simulink library "Linkage_Uprights"  (R2025a)
settings: Solver=VariableStepAuto  StartTime=0.0  StopTime=10.0  RelTol=1e-3
undefined symbols (not defined in the file): acamber, atoe, axle_len, axle_mass, axle_whlc_to_bearing, clr_axle, clr_conn_upr, clr_upr, hp_out_c_la, hp_out_f_la, hp_out_f_ua, hp_out_la, hp_out_r_la, hp_out_r_ua, hp_out_ua, hp_pushrod_out, hp_spr_bot, hp_upr_arb, hp_upr_cg, hp_upr_rod, hp_upr_wc, opc_axle, opc_conn_upr, opc_upr, radius_axle, radius_upr, size_conn_upr, upr_mass, whl_init_spd, X, Y, Z
libraries: sm_lib x147, Suspension_Utilities x50, fl_lib x9, nesl_utility x9
(part 3 of 5)

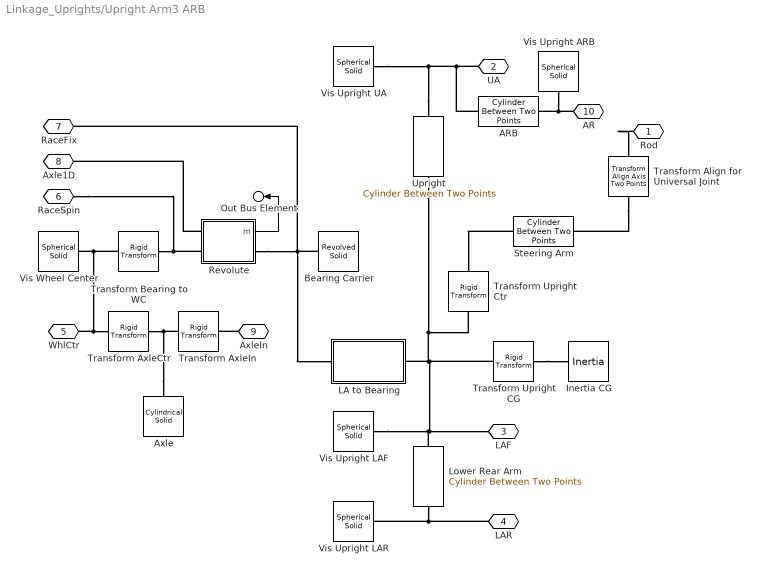
== system Linkage_Uprights/Upright Arm3 ARB ==
  ARB : Suspension_Utilities/Cylinder Between Two Points  hp_b=hp_ua_out.*rhs_hp  hp_f=hp_upr_arb.*rhs_hp  Mass=0  clr_solid=clr_upr  opc_solid=opc_upr  rad_solid=radius_upr
  Axle : sm_lib/Body Elements/Cylindrical Solid  CylinderRadius=radius_axle  CylinderRadiusUnits=m  CylinderLength=axle_len  CylinderLengthUnits=m  ExportEntireGeometry=off  InertiaType=CalculateFromGeometry  BasedOnType=Mass  Density=7000  DensityUnits=kg/m^3  Mass=axle_mass  MassUnits=kg  CenterOfMass=[0 0 0]  CenterOfMassUnits=m  MomentsOfInertia=[1 1 1]  MomentsOfInertiaUnits=kg*m^2  ProductsOfInertia=[0 0 0]  ProductsOfInertiaUnits=kg*m^2  GraphicType=FromGeometry  MarkerShape=Sphere  MarkerSize=10  GraphicVisPropType=SimpleVisualProperties  GraphicDiffuseColor=clr_axle  GraphicOpacity=opc_axle  GraphicSpecularColor=[0.5 0.5 0.5 1.0]  GraphicAmbientColor=[0.15 0.15 0.15 1.0]  GraphicEmissiveColor=[0.0 0.0 0.0 1.0]  GraphicShininess=75  DoExposeReferenceFrame=on  SerializedFrames=<Frames/>
  Bearing Carrier : sm_lib/Body Elements/Revolved Solid  RevolutionCrossSection=[1.2 0.5;1.1 0.5;1.1 -0.5;1.2 -0.5].*[radius_axle 0.05]  RevolutionCrossSectionUnits=m  RevolutionExtent=Full  RevolutionAngle=180  RevolutionAngleUnits=deg  ExportConvexHullGeometry=off  InertiaType=CalculateFromGeometry  BasedOnType=Density  Density=1000  DensityUnits=kg/m^3  Mass=1  MassUnits=kg  CenterOfMass=[0 0 0]  CenterOfMassUnits=m  MomentsOfInertia=[1 1 1]  MomentsOfInertiaUnits=kg*m^2  ProductsOfInertia=[0 0 0]  ProductsOfInertiaUnits=kg*m^2  GraphicType=FromGeometry  MarkerShape=Sphere  MarkerSize=10  GraphicVisPropType=SimpleVisualProperties  GraphicDiffuseColor=clr_upr  GraphicOpacity=0.5  GraphicSpecularColor=[0.5 0.5 0.5 1.0]  GraphicAmbientColor=[0.15 0.15 0.15 1.0]  GraphicEmissiveColor=[0.0 0.0 0.0 1.0]  GraphicShininess=75  DoExposeReferenceFrame=on  SerializedFrames=<Frames/>
  Inertia CG : sm_lib/Body Elements/Inertia  InertiaType=PointMass  Mass=upr_mass  MassUnits=kg  CenterOfMass=[0 0 0]  CenterOfMassUnits=m  MomentsOfInertia=[1 1 1]  MomentsOfInertiaUnits=kg*m^2  ProductsOfInertia=[0 0 0]  ProductsOfInertiaUnits=kg*m^2  GraphicType=Marker  MarkerShape=Inertia  MarkerSize=20  GraphicVisPropType=SimpleVisualProperties  GraphicDiffuseColor=[0.5 0.5 0.5]  GraphicOpacity=0  GraphicSpecularColor=[0.5 0.5 0.5 1.0]  GraphicAmbientColor=[0.15 0.15 0.15 1.0]  GraphicEmissiveColor=[0.0 0.0 0.0 1.0]  GraphicShininess=75
  LA to Bearing : Subsystem
  Lower Rear Arm : Suspension_Utilities/Cylinder Between Two Points  hp_b=hp_laf_out.*rhs_hp  hp_f=hp_lar_out.*rhs_hp  Mass=0  clr_solid=clr_upr  opc_solid=opc_upr  rad_solid=radius_upr
  Revolute : Subsystem  mask(Revolute Joint with 1D connections){whl_init_spd_jnt=whl_init_spd_upr}
      mask prompts: whl_init_spd_jnt "Initial Wheel Speed (rad/s)"
      mask help: Multibody Revolute Joint with connection to 1D mechanical network. Specify initial speed of Revolute Joint.
      mask Display: image('sm_car_variant_revolute.png')
  Steering Arm : Suspension_Utilities/Cylinder Between Two Points  hp_b=(hp_laf_out+0.5*(hp_ua_out-hp_laf_out)).*rhs_hp  hp_f=hp_upr_rod.*rhs_hp  Mass=0  clr_solid=clr_upr  opc_solid=opc_upr  rad_solid=radius_upr
  Transform Align for Universal Joint : Suspension_Utilities/Transform Align Axis Two Points  hp_b=(hp_laf_out+0.5*(hp_ua_out-hp_laf_out)).*rhs_hp  hp_t=hp_upr_rod.*rhs_hp  popup_f_axis=+Z
  Transform AxleCtr : sm_lib/Frames and Transforms/Rigid Transform  RotationMethod=None  FollAlignAxisA=+X  BaseAlignAxisA=+Y  FollAlignAxisB=+Y  BaseAlignAxisB=+Z  RotationStandardAxis=+Z  RotationAngle=0  RotationAngleUnits=deg  RotationArbitraryAxis=[0 0 1]  RotationSequenceAxes=FollowerAxes  RotationSequence=XYX  RotationSequenceAngles=[0 0 0]  RotationSequenceAnglesUnits=deg  RotationMatrix=[1 0 0; 0 1 0; 0 0 1]  Quaternion=[1 0 0 0]  TranslationMethod=StandardAxis  TranslationCartesianOffset=[0 0 0]  TranslationCartesianOffsetUnits=m  TranslationStandardAxis=-Z  TranslationStandardOffset=axle_len*rhs_upr/2  TranslationStandardOffsetUnits=m  TranslationROffset=0  TranslationROffsetUnits=m  TranslationThetaOffset=0  TranslationThetaOffsetUnits=deg  TranslationZOffset=0  TranslationZOffsetUnits=m
  Transform AxleIn : sm_lib/Frames and Transforms/Rigid Transform  RotationMethod=None  FollAlignAxisA=+X  BaseAlignAxisA=+Y  FollAlignAxisB=+Y  BaseAlignAxisB=+Z  RotationStandardAxis=+Z  RotationAngle=0  RotationAngleUnits=deg  RotationArbitraryAxis=[0 0 1]  RotationSequenceAxes=FollowerAxes  RotationSequence=XYX  RotationSequenceAngles=[0 0 0]  RotationSequenceAnglesUnits=deg  RotationMatrix=[1 0 0; 0 1 0; 0 0 1]  Quaternion=[1 0 0 0]  TranslationMethod=StandardAxis  TranslationCartesianOffset=[0 0 0]  TranslationCartesianOffsetUnits=m  TranslationStandardAxis=-Z  TranslationStandardOffset=axle_len*rhs_upr/2  TranslationStandardOffsetUnits=m  TranslationROffset=0  TranslationROffsetUnits=m  TranslationThetaOffset=0  TranslationThetaOffsetUnits=deg  TranslationZOffset=0  TranslationZOffsetUnits=m
  Transform Bearing to WC : sm_lib/Frames and Transforms/Rigid Transform  RotationMethod=None  FollAlignAxisA=+X  BaseAlignAxisA=+Y  FollAlignAxisB=+Y  BaseAlignAxisB=+Z  RotationStandardAxis=+Z  RotationAngle=0  RotationAngleUnits=deg  RotationArbitraryAxis=[0 0 1]  RotationSequenceAxes=FollowerAxes  RotationSequence=XYX  RotationSequenceAngles=[0 0 0]  RotationSequenceAnglesUnits=deg  RotationMatrix=[1 0 0; 0 1 0; 0 0 1]  Quaternion=[1 0 0 0]  TranslationMethod=StandardAxis  TranslationCartesianOffset=[0 0 0]  TranslationCartesianOffsetUnits=m  TranslationStandardAxis=+Z  TranslationStandardOffset=axle_whlc_to_bearing*rhs_upr  TranslationStandardOffsetUnits=m  TranslationROffset=0  TranslationROffsetUnits=m  TranslationThetaOffset=0  TranslationThetaOffsetUnits=deg  TranslationZOffset=0  TranslationZOffsetUnits=m
  Transform Upright CG : sm_lib/Frames and Transforms/Rigid Transform  RotationMethod=None  FollAlignAxisA=+X  BaseAlignAxisA=+Y  FollAlignAxisB=+Y  BaseAlignAxisB=+Z  RotationStandardAxis=+Z  RotationAngle=0.0  RotationAngleUnits=deg  RotationArbitraryAxis=[0 0 1]  RotationSequenceAxes=FollowerAxes  RotationSequence=XYX  RotationSequenceAngles=[0 0 0]  RotationSequenceAnglesUnits=deg  RotationMatrix=[1 0 0; 0 1 0; 0 0 1]  Quaternion=[1 0 0 0]  TranslationMethod=Cartesian  TranslationCartesianOffset=(hp_upr_cg-hp_laf_out) .* [1, rhs_upr, 1]  TranslationCartesianOffsetUnits=m  TranslationStandardAxis=+Z  TranslationStandardOffset=0  TranslationStandardOffsetUnits=m  TranslationROffset=0  TranslationROffsetUnits=m  TranslationThetaOffset=0  TranslationThetaOffsetUnits=deg  TranslationZOffset=0  TranslationZOffsetUnits=m
  Transform Upright Ctr : sm_lib/Frames and Transforms/Rigid Transform  RotationMethod=None  FollAlignAxisA=+X  BaseAlignAxisA=+Y  FollAlignAxisB=+Y  BaseAlignAxisB=+Z  RotationStandardAxis=+Z  RotationAngle=0.0  RotationAngleUnits=deg  RotationArbitraryAxis=[0 0 1]  RotationSequenceAxes=FollowerAxes  RotationSequence=XYX  RotationSequenceAngles=[0 0 0]  RotationSequenceAnglesUnits=deg  RotationMatrix=[1 0 0; 0 1 0; 0 0 1]  Quaternion=[1 0 0 0]  TranslationMethod=Cartesian  TranslationCartesianOffset=0.5*(hp_ua_out-hp_laf_out).*rhs_hp  TranslationCartesianOffsetUnits=m  TranslationStandardAxis=+Z  TranslationStandardOffset=0  TranslationStandardOffsetUnits=m  TranslationROffset=0  TranslationROffsetUnits=m  TranslationThetaOffset=0  TranslationThetaOffsetUnits=deg  TranslationZOffset=0  TranslationZOffsetUnits=m
  Upright : Suspension_Utilities/Cylinder Between Two Points  hp_b=hp_laf_out.*rhs_hp  hp_f=hp_ua_out.*rhs_hp  Mass=0  clr_solid=clr_upr  opc_solid=opc_upr  rad_solid=radius_upr
  Vis Upright ARB : sm_lib/Body Elements/Spherical Solid  SphereRadius=size_conn_upr  SphereRadiusUnits=m  ExportEntireGeometry=off  InertiaType=PointMass  BasedOnType=Density  Density=0  DensityUnits=kg/m^3  Mass=0  MassUnits=kg  CenterOfMass=[0 0 0]  CenterOfMassUnits=m  MomentsOfInertia=[1 1 1]  MomentsOfInertiaUnits=kg*m^2  ProductsOfInertia=[0 0 0]  ProductsOfInertiaUnits=kg*m^2  GraphicType=FromGeometry  MarkerShape=Sphere  MarkerSize=10  GraphicVisPropType=SimpleVisualProperties  GraphicDiffuseColor=clr_conn_upr  GraphicOpacity=opc_conn_upr  GraphicSpecularColor=[0.5 0.5 0.5 1.0]  GraphicAmbientColor=[0.15 0.15 0.15 1.0]  GraphicEmissiveColor=[0.0 0.0 0.0 1.0]  GraphicShininess=75  DoExposeReferenceFrame=on  SerializedFrames=<Frames/>
  Vis Upright LAF : sm_lib/Body Elements/Spherical Solid  SphereRadius=size_conn_upr  SphereRadiusUnits=m  ExportEntireGeometry=off  InertiaType=PointMass  BasedOnType=Density  Density=0  DensityUnits=kg/m^3  Mass=0  MassUnits=kg  CenterOfMass=[0 0 0]  CenterOfMassUnits=m  MomentsOfInertia=[1 1 1]  MomentsOfInertiaUnits=kg*m^2  ProductsOfInertia=[0 0 0]  ProductsOfInertiaUnits=kg*m^2  GraphicType=FromGeometry  MarkerShape=Sphere  MarkerSize=10  GraphicVisPropType=SimpleVisualProperties  GraphicDiffuseColor=clr_conn_upr  GraphicOpacity=opc_conn_upr  GraphicSpecularColor=[0.5 0.5 0.5 1.0]  GraphicAmbientColor=[0.15 0.15 0.15 1.0]  GraphicEmissiveColor=[0.0 0.0 0.0 1.0]  GraphicShininess=75  DoExposeReferenceFrame=on  SerializedFrames=<Frames/>
  Vis Upright LAR : sm_lib/Body Elements/Spherical Solid  SphereRadius=size_conn_upr  SphereRadiusUnits=m  ExportEntireGeometry=off  InertiaType=PointMass  BasedOnType=Density  Density=0  DensityUnits=kg/m^3  Mass=0  MassUnits=kg  CenterOfMass=[0 0 0]  CenterOfMassUnits=m  MomentsOfInertia=[1 1 1]  MomentsOfInertiaUnits=kg*m^2  ProductsOfInertia=[0 0 0]  ProductsOfInertiaUnits=kg*m^2  GraphicType=FromGeometry  MarkerShape=Sphere  MarkerSize=10  GraphicVisPropType=SimpleVisualProperties  GraphicDiffuseColor=clr_conn_upr  GraphicOpacity=opc_conn_upr  GraphicSpecularColor=[0.5 0.5 0.5 1.0]  GraphicAmbientColor=[0.15 0.15 0.15 1.0]  GraphicEmissiveColor=[0.0 0.0 0.0 1.0]  GraphicShininess=75  DoExposeReferenceFrame=on  SerializedFrames=<Frames/>
  Vis Upright UA : sm_lib/Body Elements/Spherical Solid  SphereRadius=size_conn_upr  SphereRadiusUnits=m  ExportEntireGeometry=off  InertiaType=PointMass  BasedOnType=Density  Density=0  DensityUnits=kg/m^3  Mass=0  MassUnits=kg  CenterOfMass=[0 0 0]  CenterOfMassUnits=m  MomentsOfInertia=[1 1 1]  MomentsOfInertiaUnits=kg*m^2  ProductsOfInertia=[0 0 0]  ProductsOfInertiaUnits=kg*m^2  GraphicType=FromGeometry  MarkerShape=Sphere  MarkerSize=10  GraphicVisPropType=SimpleVisualProperties  GraphicDiffuseColor=clr_conn_upr  GraphicOpacity=opc_conn_upr  GraphicSpecularColor=[0.5 0.5 0.5 1.0]  GraphicAmbientColor=[0.15 0.15 0.15 1.0]  GraphicEmissiveColor=[0.0 0.0 0.0 1.0]  GraphicShininess=75  DoExposeReferenceFrame=on  SerializedFrames=<Frames/>
  Vis Wheel Center : sm_lib/Body Elements/Spherical Solid  SphereRadius=size_conn_upr  SphereRadiusUnits=m  ExportEntireGeometry=off  InertiaType=PointMass  BasedOnType=Density  Density=0  DensityUnits=kg/m^3  Mass=0  MassUnits=kg  CenterOfMass=[0 0 0]  CenterOfMassUnits=m  MomentsOfInertia=[1 1 1]  MomentsOfInertiaUnits=kg*m^2  ProductsOfInertia=[0 0 0]  ProductsOfInertiaUnits=kg*m^2  GraphicType=FromGeometry  MarkerShape=Sphere  MarkerSize=10  GraphicVisPropType=SimpleVisualProperties  GraphicDiffuseColor=clr_conn_upr  GraphicOpacity=opc_conn_upr  GraphicSpecularColor=[0.5 0.5 0.5 1.0]  GraphicAmbientColor=[0.15 0.15 0.15 1.0]  GraphicEmissiveColor=[0.0 0.0 0.0 1.0]  GraphicShininess=75  DoExposeReferenceFrame=on  SerializedFrames=<Frames/>
  Rod : PMIOPort  Side=Right
  UA : PMIOPort  Port=2  Side=Right
  LAF : PMIOPort  Port=3  Side=Right
  LAR : PMIOPort  Port=4  Side=Right
  WhlCtr : PMIOPort  Port=5  Side=Left
  RaceSpin : PMIOPort  Port=6  Side=Left
  RaceFix : PMIOPort  Port=7  Side=Left
  Axle1D : PMIOPort  Port=8  Side=Left
  AxleIn : PMIOPort  Port=9  Side=Left
  AR : PMIOPort  Port=10  Side=Right
  Out Bus Element : Outport  VectorParamsAs1DForOutWhenUnconnected=off  PortName=m  Element=Bearing
  wires:
  Revolute/1(m) -> Out Bus Element/1
  connections:
  AxleIn/RConn1 -- Transform AxleIn/RConn1
  Revolute/LConn1 -- Axle1D/RConn1
  Vis Wheel Center/RConn1 -- Transform AxleCtr/LConn1 -- WhlCtr/RConn1 -- Transform Bearing to WC/RConn1
  RaceSpin/RConn1 -- Revolute/LConn2 -- Transform Bearing to WC/LConn1
  Bearing Carrier/RConn1 -- Revolute/RConn1 -- RaceFix/RConn1 -- LA to Bearing/LConn1
  Axle/RConn1 -- Transform AxleIn/LConn1 -- Transform AxleCtr/RConn1
  Lower Rear Arm/LConn1 -- Transform Upright CG/LConn1 -- LA to Bearing/RConn1 -- Transform Upright Ctr/LConn1 -- Upright/LConn1 -- LAF/RConn1 -- Vis Upright LAF/RConn1
  Upright/RConn1 -- ARB/LConn1 -- UA/RConn1 -- Vis Upright UA/RConn1
  Transform Upright CG/RConn1 -- Inertia CG/RConn1
  Steering Arm/LConn1 -- Transform Upright Ctr/RConn1
  Rod/RConn1 -- Transform Align for Universal Joint/RConn1
  Transform Align for Universal Joint/LConn1 -- Steering Arm/RConn1
  LAR/RConn1 -- Lower Rear Arm/RConn1 -- Vis Upright LAR/RConn1
  AR/RConn1 -- ARB/RConn1 -- Vis Upright ARB/RConn1

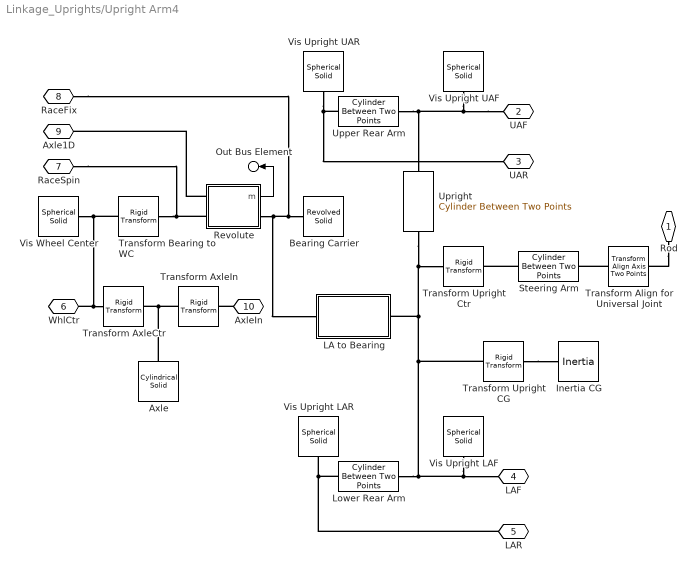
== system Linkage_Uprights/Upright Arm4 ==
  Axle : sm_lib/Body Elements/Cylindrical Solid  CylinderRadius=radius_axle  CylinderRadiusUnits=m  CylinderLength=axle_len  CylinderLengthUnits=m  ExportEntireGeometry=off  InertiaType=CalculateFromGeometry  BasedOnType=Mass  Density=7000  DensityUnits=kg/m^3  Mass=axle_mass  MassUnits=kg  CenterOfMass=[0 0 0]  CenterOfMassUnits=m  MomentsOfInertia=[1 1 1]  MomentsOfInertiaUnits=kg*m^2  ProductsOfInertia=[0 0 0]  ProductsOfInertiaUnits=kg*m^2  GraphicType=FromGeometry  MarkerShape=Sphere  MarkerSize=10  GraphicVisPropType=SimpleVisualProperties  GraphicDiffuseColor=clr_axle  GraphicOpacity=opc_axle  GraphicSpecularColor=[0.5 0.5 0.5 1.0]  GraphicAmbientColor=[0.15 0.15 0.15 1.0]  GraphicEmissiveColor=[0.0 0.0 0.0 1.0]  GraphicShininess=75  DoExposeReferenceFrame=on  SerializedFrames=<Frames/>
  Bearing Carrier : sm_lib/Body Elements/Revolved Solid  RevolutionCrossSection=[1.2 0.5;1.1 0.5;1.1 -0.5;1.2 -0.5].*[radius_axle 0.05]  RevolutionCrossSectionUnits=m  RevolutionExtent=Full  RevolutionAngle=180  RevolutionAngleUnits=deg  ExportConvexHullGeometry=off  InertiaType=CalculateFromGeometry  BasedOnType=Density  Density=1000  DensityUnits=kg/m^3  Mass=1  MassUnits=kg  CenterOfMass=[0 0 0]  CenterOfMassUnits=m  MomentsOfInertia=[1 1 1]  MomentsOfInertiaUnits=kg*m^2  ProductsOfInertia=[0 0 0]  ProductsOfInertiaUnits=kg*m^2  GraphicType=FromGeometry  MarkerShape=Sphere  MarkerSize=10  GraphicVisPropType=SimpleVisualProperties  GraphicDiffuseColor=clr_upr  GraphicOpacity=0.5  GraphicSpecularColor=[0.5 0.5 0.5 1.0]  GraphicAmbientColor=[0.15 0.15 0.15 1.0]  GraphicEmissiveColor=[0.0 0.0 0.0 1.0]  GraphicShininess=75  DoExposeReferenceFrame=on  SerializedFrames=<Frames/>
  Inertia CG : sm_lib/Body Elements/Inertia  InertiaType=PointMass  Mass=upr_mass  MassUnits=kg  CenterOfMass=[0 0 0]  CenterOfMassUnits=m  MomentsOfInertia=[1 1 1]  MomentsOfInertiaUnits=kg*m^2  ProductsOfInertia=[0 0 0]  ProductsOfInertiaUnits=kg*m^2  GraphicType=Marker  MarkerShape=Inertia  MarkerSize=20  GraphicVisPropType=SimpleVisualProperties  GraphicDiffuseColor=[0.5 0.5 0.5]  GraphicOpacity=0  GraphicSpecularColor=[0.5 0.5 0.5 1.0]  GraphicAmbientColor=[0.15 0.15 0.15 1.0]  GraphicEmissiveColor=[0.0 0.0 0.0 1.0]  GraphicShininess=75
  LA to Bearing : Subsystem
  Lower Rear Arm : Suspension_Utilities/Cylinder Between Two Points  hp_b=hp_laf_out.*rhs_hp  hp_f=hp_lar_out.*rhs_hp  Mass=0  clr_solid=clr_upr  opc_solid=opc_upr  rad_solid=radius_upr
  Revolute : Subsystem  mask(Revolute Joint with 1D connections){whl_init_spd_jnt=whl_init_spd_upr}
      mask prompts: whl_init_spd_jnt "Initial Wheel Speed (rad/s)"
      mask help: Multibody Revolute Joint with connection to 1D mechanical network. Specify initial speed of Revolute Joint.
      mask Display: image('sm_car_variant_revolute.png')
  Steering Arm : Suspension_Utilities/Cylinder Between Two Points  hp_b=(hp_laf_out+0.5*(hp_uaf_out-hp_laf_out)).*rhs_hp  hp_f=hp_upr_rod.*rhs_hp  Mass=0  clr_solid=clr_upr  opc_solid=opc_upr  rad_solid=radius_upr
  Transform Align for Universal Joint : Suspension_Utilities/Transform Align Axis Two Points  hp_b=(hp_laf_out+0.5*(hp_uaf_out-hp_laf_out)).*rhs_hp  hp_t=hp_upr_rod.*rhs_hp  popup_f_axis=+Z
  Transform AxleCtr : sm_lib/Frames and Transforms/Rigid Transform  RotationMethod=None  FollAlignAxisA=+X  BaseAlignAxisA=+Y  FollAlignAxisB=+Y  BaseAlignAxisB=+Z  RotationStandardAxis=+Z  RotationAngle=0  RotationAngleUnits=deg  RotationArbitraryAxis=[0 0 1]  RotationSequenceAxes=FollowerAxes  RotationSequence=XYX  RotationSequenceAngles=[0 0 0]  RotationSequenceAnglesUnits=deg  RotationMatrix=[1 0 0; 0 1 0; 0 0 1]  Quaternion=[1 0 0 0]  TranslationMethod=StandardAxis  TranslationCartesianOffset=[0 0 0]  TranslationCartesianOffsetUnits=m  TranslationStandardAxis=-Z  TranslationStandardOffset=axle_len*rhs_upr/2  TranslationStandardOffsetUnits=m  TranslationROffset=0  TranslationROffsetUnits=m  TranslationThetaOffset=0  TranslationThetaOffsetUnits=deg  TranslationZOffset=0  TranslationZOffsetUnits=m
  Transform AxleIn : sm_lib/Frames and Transforms/Rigid Transform  RotationMethod=None  FollAlignAxisA=+X  BaseAlignAxisA=+Y  FollAlignAxisB=+Y  BaseAlignAxisB=+Z  RotationStandardAxis=+Z  RotationAngle=0  RotationAngleUnits=deg  RotationArbitraryAxis=[0 0 1]  RotationSequenceAxes=FollowerAxes  RotationSequence=XYX  RotationSequenceAngles=[0 0 0]  RotationSequenceAnglesUnits=deg  RotationMatrix=[1 0 0; 0 1 0; 0 0 1]  Quaternion=[1 0 0 0]  TranslationMethod=StandardAxis  TranslationCartesianOffset=[0 0 0]  TranslationCartesianOffsetUnits=m  TranslationStandardAxis=-Z  TranslationStandardOffset=axle_len*rhs_upr/2  TranslationStandardOffsetUnits=m  TranslationROffset=0  TranslationROffsetUnits=m  TranslationThetaOffset=0  TranslationThetaOffsetUnits=deg  TranslationZOffset=0  TranslationZOffsetUnits=m
  Transform Bearing to WC : sm_lib/Frames and Transforms/Rigid Transform  RotationMethod=None  FollAlignAxisA=+X  BaseAlignAxisA=+Y  FollAlignAxisB=+Y  BaseAlignAxisB=+Z  RotationStandardAxis=+Z  RotationAngle=0  RotationAngleUnits=deg  RotationArbitraryAxis=[0 0 1]  RotationSequenceAxes=FollowerAxes  RotationSequence=XYX  RotationSequenceAngles=[0 0 0]  RotationSequenceAnglesUnits=deg  RotationMatrix=[1 0 0; 0 1 0; 0 0 1]  Quaternion=[1 0 0 0]  TranslationMethod=StandardAxis  TranslationCartesianOffset=[0 0 0]  TranslationCartesianOffsetUnits=m  TranslationStandardAxis=+Z  TranslationStandardOffset=axle_whlc_to_bearing*rhs_upr  TranslationStandardOffsetUnits=m  TranslationROffset=0  TranslationROffsetUnits=m  TranslationThetaOffset=0  TranslationThetaOffsetUnits=deg  TranslationZOffset=0  TranslationZOffsetUnits=m
  Transform Upright CG : sm_lib/Frames and Transforms/Rigid Transform  RotationMethod=None  FollAlignAxisA=+X  BaseAlignAxisA=+Y  FollAlignAxisB=+Y  BaseAlignAxisB=+Z  RotationStandardAxis=+Z  RotationAngle=0.0  RotationAngleUnits=deg  RotationArbitraryAxis=[0 0 1]  RotationSequenceAxes=FollowerAxes  RotationSequence=XYX  RotationSequenceAngles=[0 0 0]  RotationSequenceAnglesUnits=deg  RotationMatrix=[1 0 0; 0 1 0; 0 0 1]  Quaternion=[1 0 0 0]  TranslationMethod=Cartesian  TranslationCartesianOffset=(hp_upr_cg-hp_laf_out) .* [1, rhs_upr, 1]  TranslationCartesianOffsetUnits=m  TranslationStandardAxis=+Z  TranslationStandardOffset=0  TranslationStandardOffsetUnits=m  TranslationROffset=0  TranslationROffsetUnits=m  TranslationThetaOffset=0  TranslationThetaOffsetUnits=deg  TranslationZOffset=0  TranslationZOffsetUnits=m
  Transform Upright Ctr : sm_lib/Frames and Transforms/Rigid Transform  RotationMethod=None  FollAlignAxisA=+X  BaseAlignAxisA=+Y  FollAlignAxisB=+Y  BaseAlignAxisB=+Z  RotationStandardAxis=+Z  RotationAngle=0.0  RotationAngleUnits=deg  RotationArbitraryAxis=[0 0 1]  RotationSequenceAxes=FollowerAxes  RotationSequence=XYX  RotationSequenceAngles=[0 0 0]  RotationSequenceAnglesUnits=deg  RotationMatrix=[1 0 0; 0 1 0; 0 0 1]  Quaternion=[1 0 0 0]  TranslationMethod=Cartesian  TranslationCartesianOffset=0.5*(hp_uaf_out-hp_laf_out).*rhs_hp  TranslationCartesianOffsetUnits=m  TranslationStandardAxis=+Z  TranslationStandardOffset=0  TranslationStandardOffsetUnits=m  TranslationROffset=0  TranslationROffsetUnits=m  TranslationThetaOffset=0  TranslationThetaOffsetUnits=deg  TranslationZOffset=0  TranslationZOffsetUnits=m
  Upper Rear Arm : Suspension_Utilities/Cylinder Between Two Points  hp_b=hp_uaf_out.*rhs_hp  hp_f=hp_uar_out.*rhs_hp  Mass=0  clr_solid=clr_upr  opc_solid=opc_upr  rad_solid=radius_upr
  Upright : Suspension_Utilities/Cylinder Between Two Points  hp_b=hp_laf_out.*rhs_hp  hp_f=hp_uaf_out.*rhs_hp  Mass=0  clr_solid=clr_upr  opc_solid=opc_upr  rad_solid=radius_upr
  Vis Wheel Center : sm_lib/Body Elements/Spherical Solid  SphereRadius=size_conn_upr  SphereRadiusUnits=m  ExportEntireGeometry=off  InertiaType=PointMass  BasedOnType=Density  Density=0  DensityUnits=kg/m^3  Mass=0  MassUnits=kg  CenterOfMass=[0 0 0]  CenterOfMassUnits=m  MomentsOfInertia=[1 1 1]  MomentsOfInertiaUnits=kg*m^2  ProductsOfInertia=[0 0 0]  ProductsOfInertiaUnits=kg*m^2  GraphicType=FromGeometry  MarkerShape=Sphere  MarkerSize=10  GraphicVisPropType=SimpleVisualProperties  GraphicDiffuseColor=clr_conn_upr  GraphicOpacity=opc_conn_upr  GraphicSpecularColor=[0.5 0.5 0.5 1.0]  GraphicAmbientColor=[0.15 0.15 0.15 1.0]  GraphicEmissiveColor=[0.0 0.0 0.0 1.0]  GraphicShininess=75  DoExposeReferenceFrame=on  SerializedFrames=<Frames/>
  Vis Upright LAF : sm_lib/Body Elements/Spherical Solid  SphereRadius=size_conn_upr  SphereRadiusUnits=m  ExportEntireGeometry=off  InertiaType=PointMass  BasedOnType=Density  Density=0  DensityUnits=kg/m^3  Mass=0  MassUnits=kg  CenterOfMass=[0 0 0]  CenterOfMassUnits=m  MomentsOfInertia=[1 1 1]  MomentsOfInertiaUnits=kg*m^2  ProductsOfInertia=[0 0 0]  ProductsOfInertiaUnits=kg*m^2  GraphicType=FromGeometry  MarkerShape=Sphere  MarkerSize=10  GraphicVisPropType=SimpleVisualProperties  GraphicDiffuseColor=clr_conn_upr  GraphicOpacity=opc_conn_upr  GraphicSpecularColor=[0.5 0.5 0.5 1.0]  GraphicAmbientColor=[0.15 0.15 0.15 1.0]  GraphicEmissiveColor=[0.0 0.0 0.0 1.0]  GraphicShininess=75  DoExposeReferenceFrame=on  SerializedFrames=<Frames/>
  Vis Upright LAR : sm_lib/Body Elements/Spherical Solid  SphereRadius=size_conn_upr  SphereRadiusUnits=m  ExportEntireGeometry=off  InertiaType=PointMass  BasedOnType=Density  Density=0  DensityUnits=kg/m^3  Mass=0  MassUnits=kg  CenterOfMass=[0 0 0]  CenterOfMassUnits=m  MomentsOfInertia=[1 1 1]  MomentsOfInertiaUnits=kg*m^2  ProductsOfInertia=[0 0 0]  ProductsOfInertiaUnits=kg*m^2  GraphicType=FromGeometry  MarkerShape=Sphere  MarkerSize=10  GraphicVisPropType=SimpleVisualProperties  GraphicDiffuseColor=clr_conn_upr  GraphicOpacity=opc_conn_upr  GraphicSpecularColor=[0.5 0.5 0.5 1.0]  GraphicAmbientColor=[0.15 0.15 0.15 1.0]  GraphicEmissiveColor=[0.0 0.0 0.0 1.0]  GraphicShininess=75  DoExposeReferenceFrame=on  SerializedFrames=<Frames/>
  Vis Upright UAF : sm_lib/Body Elements/Spherical Solid  SphereRadius=size_conn_upr  SphereRadiusUnits=m  ExportEntireGeometry=off  InertiaType=PointMass  BasedOnType=Density  Density=0  DensityUnits=kg/m^3  Mass=0  MassUnits=kg  CenterOfMass=[0 0 0]  CenterOfMassUnits=m  MomentsOfInertia=[1 1 1]  MomentsOfInertiaUnits=kg*m^2  ProductsOfInertia=[0 0 0]  ProductsOfInertiaUnits=kg*m^2  GraphicType=FromGeometry  MarkerShape=Sphere  MarkerSize=10  GraphicVisPropType=SimpleVisualProperties  GraphicDiffuseColor=clr_conn_upr  GraphicOpacity=opc_conn_upr  GraphicSpecularColor=[0.5 0.5 0.5 1.0]  GraphicAmbientColor=[0.15 0.15 0.15 1.0]  GraphicEmissiveColor=[0.0 0.0 0.0 1.0]  GraphicShininess=75  DoExposeReferenceFrame=on  SerializedFrames=<Frames/>
  Vis Upright UAR : sm_lib/Body Elements/Spherical Solid  SphereRadius=size_conn_upr  SphereRadiusUnits=m  ExportEntireGeometry=off  InertiaType=PointMass  BasedOnType=Density  Density=0  DensityUnits=kg/m^3  Mass=0  MassUnits=kg  CenterOfMass=[0 0 0]  CenterOfMassUnits=m  MomentsOfInertia=[1 1 1]  MomentsOfInertiaUnits=kg*m^2  ProductsOfInertia=[0 0 0]  ProductsOfInertiaUnits=kg*m^2  GraphicType=FromGeometry  MarkerShape=Sphere  MarkerSize=10  GraphicVisPropType=SimpleVisualProperties  GraphicDiffuseColor=clr_conn_upr  GraphicOpacity=opc_conn_upr  GraphicSpecularColor=[0.5 0.5 0.5 1.0]  GraphicAmbientColor=[0.15 0.15 0.15 1.0]  GraphicEmissiveColor=[0.0 0.0 0.0 1.0]  GraphicShininess=75  DoExposeReferenceFrame=on  SerializedFrames=<Frames/>
  Rod : PMIOPort  Side=Right
  UAF : PMIOPort  Port=2  Side=Right
  UAR : PMIOPort  Port=3  Side=Right
  LAF : PMIOPort  Port=4  Side=Right
  LAR : PMIOPort  Port=5  Side=Right
  WhlCtr : PMIOPort  Port=6  Side=Left
  RaceSpin : PMIOPort  Port=7  Side=Left
  RaceFix : PMIOPort  Port=8  Side=Left
  Axle1D : PMIOPort  Port=9  Side=Left
  AxleIn : PMIOPort  Port=10  Side=Left
  Out Bus Element : Outport  VectorParamsAs1DForOutWhenUnconnected=off  PortName=m  Element=Upright
  wires:
  Revolute/1(m) -> Out Bus Element/1
  connections:
  Vis Upright UAR/RConn1 -- UAR/RConn1 -- Upper Rear Arm/RConn1
  Lower Rear Arm/RConn1 -- LAR/RConn1 -- Vis Upright LAR/RConn1
  Transform Align for Universal Joint/LConn1 -- Steering Arm/RConn1
  Rod/RConn1 -- Transform Align for Universal Joint/RConn1
  Steering Arm/LConn1 -- Transform Upright Ctr/RConn1
  Transform Upright CG/RConn1 -- Inertia CG/RConn1
  UAF/RConn1 -- Upper Rear Arm/LConn1 -- Upright/RConn1 -- Vis Upright UAF/RConn1
  Transform Bearing to WC/LConn1 -- Revolute/LConn2 -- RaceSpin/RConn1
  Vis Wheel Center/RConn1 -- Transform Bearing to WC/RConn1 -- Transform AxleCtr/LConn1 -- WhlCtr/RConn1
  Axle/RConn1 -- Transform AxleIn/LConn1 -- Transform AxleCtr/RConn1
  Revolute/LConn1 -- Axle1D/RConn1
  Vis Upright LAF/RConn1 -- Transform Upright Ctr/LConn1 -- Upright/LConn1 -- LA to Bearing/RConn1 -- Transform Upright CG/LConn1 -- Lower Rear Arm/LConn1 -- LAF/RConn1
  RaceFix/RConn1 -- Revolute/RConn1 -- LA to Bearing/LConn1 -- Bearing Carrier/RConn1
  AxleIn/RConn1 -- Transform AxleIn/RConn1

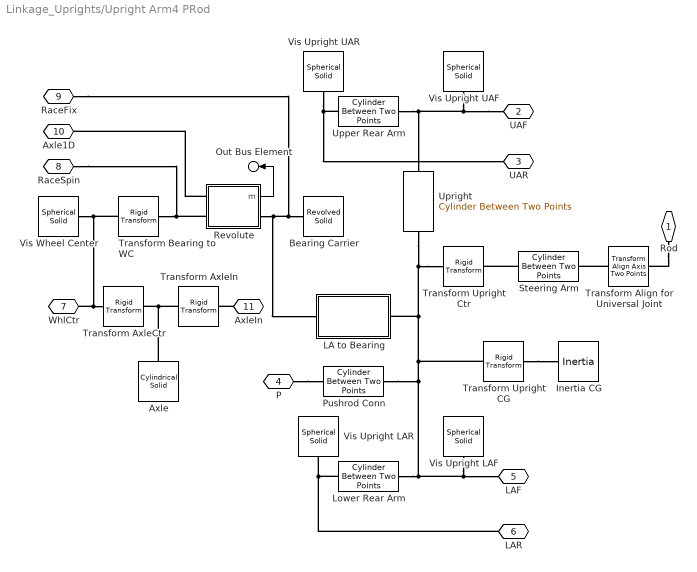
== system Linkage_Uprights/Upright Arm4 PRod ==
  Axle : sm_lib/Body Elements/Cylindrical Solid  CylinderRadius=radius_axle  CylinderRadiusUnits=m  CylinderLength=axle_len  CylinderLengthUnits=m  ExportEntireGeometry=off  InertiaType=CalculateFromGeometry  BasedOnType=Mass  Density=7000  DensityUnits=kg/m^3  Mass=axle_mass  MassUnits=kg  CenterOfMass=[0 0 0]  CenterOfMassUnits=m  MomentsOfInertia=[1 1 1]  MomentsOfInertiaUnits=kg*m^2  ProductsOfInertia=[0 0 0]  ProductsOfInertiaUnits=kg*m^2  GraphicType=FromGeometry  MarkerShape=Sphere  MarkerSize=10  GraphicVisPropType=SimpleVisualProperties  GraphicDiffuseColor=clr_axle  GraphicOpacity=opc_axle  GraphicSpecularColor=[0.5 0.5 0.5 1.0]  GraphicAmbientColor=[0.15 0.15 0.15 1.0]  GraphicEmissiveColor=[0.0 0.0 0.0 1.0]  GraphicShininess=75  DoExposeReferenceFrame=on  SerializedFrames=<Frames/>
  Bearing Carrier : sm_lib/Body Elements/Revolved Solid  RevolutionCrossSection=[1.2 0.5;1.1 0.5;1.1 -0.5;1.2 -0.5].*[radius_axle 0.05]  RevolutionCrossSectionUnits=m  RevolutionExtent=Full  RevolutionAngle=180  RevolutionAngleUnits=deg  ExportConvexHullGeometry=off  InertiaType=CalculateFromGeometry  BasedOnType=Density  Density=1000  DensityUnits=kg/m^3  Mass=1  MassUnits=kg  CenterOfMass=[0 0 0]  CenterOfMassUnits=m  MomentsOfInertia=[1 1 1]  MomentsOfInertiaUnits=kg*m^2  ProductsOfInertia=[0 0 0]  ProductsOfInertiaUnits=kg*m^2  GraphicType=FromGeometry  MarkerShape=Sphere  MarkerSize=10  GraphicVisPropType=SimpleVisualProperties  GraphicDiffuseColor=clr_upr  GraphicOpacity=0.5  GraphicSpecularColor=[0.5 0.5 0.5 1.0]  GraphicAmbientColor=[0.15 0.15 0.15 1.0]  GraphicEmissiveColor=[0.0 0.0 0.0 1.0]  GraphicShininess=75  DoExposeReferenceFrame=on  SerializedFrames=<Frames/>
  Inertia CG : sm_lib/Body Elements/Inertia  InertiaType=PointMass  Mass=upr_mass  MassUnits=kg  CenterOfMass=[0 0 0]  CenterOfMassUnits=m  MomentsOfInertia=[1 1 1]  MomentsOfInertiaUnits=kg*m^2  ProductsOfInertia=[0 0 0]  ProductsOfInertiaUnits=kg*m^2  GraphicType=Marker  MarkerShape=Inertia  MarkerSize=20  GraphicVisPropType=SimpleVisualProperties  GraphicDiffuseColor=[0.5 0.5 0.5]  GraphicOpacity=0  GraphicSpecularColor=[0.5 0.5 0.5 1.0]  GraphicAmbientColor=[0.15 0.15 0.15 1.0]  GraphicEmissiveColor=[0.0 0.0 0.0 1.0]  GraphicShininess=75
  LA to Bearing : Subsystem
  Lower Rear Arm : Suspension_Utilities/Cylinder Between Two Points  hp_b=hp_laf_out.*rhs_hp  hp_f=hp_lar_out.*rhs_hp  Mass=0  clr_solid=clr_upr  opc_solid=opc_upr  rad_solid=radius_upr
  Pushrod Conn : Suspension_Utilities/Cylinder Between Two Points  hp_b=hp_laf_out.*rhs_hp  hp_f=hp_pushrod.*rhs_hp  Mass=0  clr_solid=clr_upr  opc_solid=opc_upr  rad_solid=radius_upr
  Revolute : Subsystem  mask(Revolute Joint with 1D connections){whl_init_spd_jnt=whl_init_spd_upr}
      mask prompts: whl_init_spd_jnt "Initial Wheel Speed (rad/s)"
      mask help: Multibody Revolute Joint with connection to 1D mechanical network. Specify initial speed of Revolute Joint.
      mask Display: image('sm_car_variant_revolute.png')
  Steering Arm : Suspension_Utilities/Cylinder Between Two Points  hp_b=(hp_laf_out+0.5*(hp_uaf_out-hp_laf_out)).*rhs_hp  hp_f=hp_upr_rod.*rhs_hp  Mass=0  clr_solid=clr_upr  opc_solid=opc_upr  rad_solid=radius_upr
  Transform Align for Universal Joint : Suspension_Utilities/Transform Align Axis Two Points  hp_b=(hp_laf_out+0.5*(hp_uaf_out-hp_laf_out)).*rhs_hp  hp_t=hp_upr_rod.*rhs_hp  popup_f_axis=+Z
  Transform AxleCtr : sm_lib/Frames and Transforms/Rigid Transform  RotationMethod=None  FollAlignAxisA=+X  BaseAlignAxisA=+Y  FollAlignAxisB=+Y  BaseAlignAxisB=+Z  RotationStandardAxis=+Z  RotationAngle=0  RotationAngleUnits=deg  RotationArbitraryAxis=[0 0 1]  RotationSequenceAxes=FollowerAxes  RotationSequence=XYX  RotationSequenceAngles=[0 0 0]  RotationSequenceAnglesUnits=deg  RotationMatrix=[1 0 0; 0 1 0; 0 0 1]  Quaternion=[1 0 0 0]  TranslationMethod=StandardAxis  TranslationCartesianOffset=[0 0 0]  TranslationCartesianOffsetUnits=m  TranslationStandardAxis=-Z  TranslationStandardOffset=axle_len*rhs_upr/2  TranslationStandardOffsetUnits=m  TranslationROffset=0  TranslationROffsetUnits=m  TranslationThetaOffset=0  TranslationThetaOffsetUnits=deg  TranslationZOffset=0  TranslationZOffsetUnits=m
  Transform AxleIn : sm_lib/Frames and Transforms/Rigid Transform  RotationMethod=None  FollAlignAxisA=+X  BaseAlignAxisA=+Y  FollAlignAxisB=+Y  BaseAlignAxisB=+Z  RotationStandardAxis=+Z  RotationAngle=0  RotationAngleUnits=deg  RotationArbitraryAxis=[0 0 1]  RotationSequenceAxes=FollowerAxes  RotationSequence=XYX  RotationSequenceAngles=[0 0 0]  RotationSequenceAnglesUnits=deg  RotationMatrix=[1 0 0; 0 1 0; 0 0 1]  Quaternion=[1 0 0 0]  TranslationMethod=StandardAxis  TranslationCartesianOffset=[0 0 0]  TranslationCartesianOffsetUnits=m  TranslationStandardAxis=-Z  TranslationStandardOffset=axle_len*rhs_upr/2  TranslationStandardOffsetUnits=m  TranslationROffset=0  TranslationROffsetUnits=m  TranslationThetaOffset=0  TranslationThetaOffsetUnits=deg  TranslationZOffset=0  TranslationZOffsetUnits=m
  Transform Bearing to WC : sm_lib/Frames and Transforms/Rigid Transform  RotationMethod=None  FollAlignAxisA=+X  BaseAlignAxisA=+Y  FollAlignAxisB=+Y  BaseAlignAxisB=+Z  RotationStandardAxis=+Z  RotationAngle=0  RotationAngleUnits=deg  RotationArbitraryAxis=[0 0 1]  RotationSequenceAxes=FollowerAxes  RotationSequence=XYX  RotationSequenceAngles=[0 0 0]  RotationSequenceAnglesUnits=deg  RotationMatrix=[1 0 0; 0 1 0; 0 0 1]  Quaternion=[1 0 0 0]  TranslationMethod=StandardAxis  TranslationCartesianOffset=[0 0 0]  TranslationCartesianOffsetUnits=m  TranslationStandardAxis=+Z  TranslationStandardOffset=axle_whlc_to_bearing*rhs_upr  TranslationStandardOffsetUnits=m  TranslationROffset=0  TranslationROffsetUnits=m  TranslationThetaOffset=0  TranslationThetaOffsetUnits=deg  TranslationZOffset=0  TranslationZOffsetUnits=m
  Transform Upright CG : sm_lib/Frames and Transforms/Rigid Transform  RotationMethod=None  FollAlignAxisA=+X  BaseAlignAxisA=+Y  FollAlignAxisB=+Y  BaseAlignAxisB=+Z  RotationStandardAxis=+Z  RotationAngle=0.0  RotationAngleUnits=deg  RotationArbitraryAxis=[0 0 1]  RotationSequenceAxes=FollowerAxes  RotationSequence=XYX  RotationSequenceAngles=[0 0 0]  RotationSequenceAnglesUnits=deg  RotationMatrix=[1 0 0; 0 1 0; 0 0 1]  Quaternion=[1 0 0 0]  TranslationMethod=Cartesian  TranslationCartesianOffset=(hp_upr_cg-hp_laf_out) .* [1, rhs_upr, 1]  TranslationCartesianOffsetUnits=m  TranslationStandardAxis=+Z  TranslationStandardOffset=0  TranslationStandardOffsetUnits=m  TranslationROffset=0  TranslationROffsetUnits=m  TranslationThetaOffset=0  TranslationThetaOffsetUnits=deg  TranslationZOffset=0  TranslationZOffsetUnits=m
  Transform Upright Ctr : sm_lib/Frames and Transforms/Rigid Transform  RotationMethod=None  FollAlignAxisA=+X  BaseAlignAxisA=+Y  FollAlignAxisB=+Y  BaseAlignAxisB=+Z  RotationStandardAxis=+Z  RotationAngle=0.0  RotationAngleUnits=deg  RotationArbitraryAxis=[0 0 1]  RotationSequenceAxes=FollowerAxes  RotationSequence=XYX  RotationSequenceAngles=[0 0 0]  RotationSequenceAnglesUnits=deg  RotationMatrix=[1 0 0; 0 1 0; 0 0 1]  Quaternion=[1 0 0 0]  TranslationMethod=Cartesian  TranslationCartesianOffset=0.5*(hp_uaf_out-hp_laf_out).*rhs_hp  TranslationCartesianOffsetUnits=m  TranslationStandardAxis=+Z  TranslationStandardOffset=0  TranslationStandardOffsetUnits=m  TranslationROffset=0  TranslationROffsetUnits=m  TranslationThetaOffset=0  TranslationThetaOffsetUnits=deg  TranslationZOffset=0  TranslationZOffsetUnits=m
  Upper Rear Arm : Suspension_Utilities/Cylinder Between Two Points  hp_b=hp_uaf_out.*rhs_hp  hp_f=hp_uar_out.*rhs_hp  Mass=0  clr_solid=clr_upr  opc_solid=opc_upr  rad_solid=radius_upr
  Upright : Suspension_Utilities/Cylinder Between Two Points  hp_b=hp_laf_out.*rhs_hp  hp_f=hp_uaf_out.*rhs_hp  Mass=0  clr_solid=clr_upr  opc_solid=opc_upr  rad_solid=radius_upr
  Vis Wheel Center : sm_lib/Body Elements/Spherical Solid  SphereRadius=size_conn_upr  SphereRadiusUnits=m  ExportEntireGeometry=off  InertiaType=PointMass  BasedOnType=Density  Density=0  DensityUnits=kg/m^3  Mass=0  MassUnits=kg  CenterOfMass=[0 0 0]  CenterOfMassUnits=m  MomentsOfInertia=[1 1 1]  MomentsOfInertiaUnits=kg*m^2  ProductsOfInertia=[0 0 0]  ProductsOfInertiaUnits=kg*m^2  GraphicType=FromGeometry  MarkerShape=Sphere  MarkerSize=10  GraphicVisPropType=SimpleVisualProperties  GraphicDiffuseColor=clr_conn_upr  GraphicOpacity=opc_conn_upr  GraphicSpecularColor=[0.5 0.5 0.5 1.0]  GraphicAmbientColor=[0.15 0.15 0.15 1.0]  GraphicEmissiveColor=[0.0 0.0 0.0 1.0]  GraphicShininess=75  DoExposeReferenceFrame=on  SerializedFrames=<Frames/>
  Vis Upright LAF : sm_lib/Body Elements/Spherical Solid  SphereRadius=size_conn_upr  SphereRadiusUnits=m  ExportEntireGeometry=off  InertiaType=PointMass  BasedOnType=Density  Density=0  DensityUnits=kg/m^3  Mass=0  MassUnits=kg  CenterOfMass=[0 0 0]  CenterOfMassUnits=m  MomentsOfInertia=[1 1 1]  MomentsOfInertiaUnits=kg*m^2  ProductsOfInertia=[0 0 0]  ProductsOfInertiaUnits=kg*m^2  GraphicType=FromGeometry  MarkerShape=Sphere  MarkerSize=10  GraphicVisPropType=SimpleVisualProperties  GraphicDiffuseColor=clr_conn_upr  GraphicOpacity=opc_conn_upr  GraphicSpecularColor=[0.5 0.5 0.5 1.0]  GraphicAmbientColor=[0.15 0.15 0.15 1.0]  GraphicEmissiveColor=[0.0 0.0 0.0 1.0]  GraphicShininess=75  DoExposeReferenceFrame=on  SerializedFrames=<Frames/>
  Vis Upright LAR : sm_lib/Body Elements/Spherical Solid  SphereRadius=size_conn_upr  SphereRadiusUnits=m  ExportEntireGeometry=off  InertiaType=PointMass  BasedOnType=Density  Density=0  DensityUnits=kg/m^3  Mass=0  MassUnits=kg  CenterOfMass=[0 0 0]  CenterOfMassUnits=m  MomentsOfInertia=[1 1 1]  MomentsOfInertiaUnits=kg*m^2  ProductsOfInertia=[0 0 0]  ProductsOfInertiaUnits=kg*m^2  GraphicType=FromGeometry  MarkerShape=Sphere  MarkerSize=10  GraphicVisPropType=SimpleVisualProperties  GraphicDiffuseColor=clr_conn_upr  GraphicOpacity=opc_conn_upr  GraphicSpecularColor=[0.5 0.5 0.5 1.0]  GraphicAmbientColor=[0.15 0.15 0.15 1.0]  GraphicEmissiveColor=[0.0 0.0 0.0 1.0]  GraphicShininess=75  DoExposeReferenceFrame=on  SerializedFrames=<Frames/>
  Vis Upright UAF : sm_lib/Body Elements/Spherical Solid  SphereRadius=size_conn_upr  SphereRadiusUnits=m  ExportEntireGeometry=off  InertiaType=PointMass  BasedOnType=Density  Density=0  DensityUnits=kg/m^3  Mass=0  MassUnits=kg  CenterOfMass=[0 0 0]  CenterOfMassUnits=m  MomentsOfInertia=[1 1 1]  MomentsOfInertiaUnits=kg*m^2  ProductsOfInertia=[0 0 0]  ProductsOfInertiaUnits=kg*m^2  GraphicType=FromGeometry  MarkerShape=Sphere  MarkerSize=10  GraphicVisPropType=SimpleVisualProperties  GraphicDiffuseColor=clr_conn_upr  GraphicOpacity=opc_conn_upr  GraphicSpecularColor=[0.5 0.5 0.5 1.0]  GraphicAmbientColor=[0.15 0.15 0.15 1.0]  GraphicEmissiveColor=[0.0 0.0 0.0 1.0]  GraphicShininess=75  DoExposeReferenceFrame=on  SerializedFrames=<Frames/>
  Vis Upright UAR : sm_lib/Body Elements/Spherical Solid  SphereRadius=size_conn_upr  SphereRadiusUnits=m  ExportEntireGeometry=off  InertiaType=PointMass  BasedOnType=Density  Density=0  DensityUnits=kg/m^3  Mass=0  MassUnits=kg  CenterOfMass=[0 0 0]  CenterOfMassUnits=m  MomentsOfInertia=[1 1 1]  MomentsOfInertiaUnits=kg*m^2  ProductsOfInertia=[0 0 0]  ProductsOfInertiaUnits=kg*m^2  GraphicType=FromGeometry  MarkerShape=Sphere  MarkerSize=10  GraphicVisPropType=SimpleVisualProperties  GraphicDiffuseColor=clr_conn_upr  GraphicOpacity=opc_conn_upr  GraphicSpecularColor=[0.5 0.5 0.5 1.0]  GraphicAmbientColor=[0.15 0.15 0.15 1.0]  GraphicEmissiveColor=[0.0 0.0 0.0 1.0]  GraphicShininess=75  DoExposeReferenceFrame=on  SerializedFrames=<Frames/>
  Rod : PMIOPort  Side=Right
  UAF : PMIOPort  Port=2  Side=Right
  UAR : PMIOPort  Port=3  Side=Right
  P : PMIOPort  Port=4  Side=Right
  LAF : PMIOPort  Port=5  Side=Right
  LAR : PMIOPort  Port=6  Side=Right
  WhlCtr : PMIOPort  Port=7  Side=Left
  RaceSpin : PMIOPort  Port=8  Side=Left
  RaceFix : PMIOPort  Port=9  Side=Left
  Axle1D : PMIOPort  Port=10  Side=Left
  AxleIn : PMIOPort  Port=11  Side=Left
  Out Bus Element : Outport  VectorParamsAs1DForOutWhenUnconnected=off  PortName=m  Element=Upright
  wires:
  Revolute/1(m) -> Out Bus Element/1
  connections:
  Transform Upright Ctr/LConn1 -- Upright/LConn1 -- LA to Bearing/RConn1 -- Lower Rear Arm/LConn1 -- Vis Upright LAF/RConn1 -- LAF/RConn1 -- Pushrod Conn/LConn1 -- Transform Upright CG/LConn1
  Vis Upright UAR/RConn1 -- UAR/RConn1 -- Upper Rear Arm/RConn1
  Lower Rear Arm/RConn1 -- LAR/RConn1 -- Vis Upright LAR/RConn1
  Transform Align for Universal Joint/LConn1 -- Steering Arm/RConn1
  Rod/RConn1 -- Transform Align for Universal Joint/RConn1
  Steering Arm/LConn1 -- Transform Upright Ctr/RConn1
  Transform Upright CG/RConn1 -- Inertia CG/RConn1
  UAF/RConn1 -- Upper Rear Arm/LConn1 -- Upright/RConn1 -- Vis Upright UAF/RConn1
  Transform Bearing to WC/LConn1 -- Revolute/LConn2 -- RaceSpin/RConn1
  Vis Wheel Center/RConn1 -- Transform Bearing to WC/RConn1 -- Transform AxleCtr/LConn1 -- WhlCtr/RConn1
  Axle/RConn1 -- Transform AxleIn/LConn1 -- Transform AxleCtr/RConn1
  Revolute/LConn1 -- Axle1D/RConn1
  P/RConn1 -- Pushrod Conn/RConn1
  RaceFix/RConn1 -- Revolute/RConn1 -- LA to Bearing/LConn1 -- Bearing Carrier/RConn1
  AxleIn/RConn1 -- Transform AxleIn/RConn1
